simulink model "das_evolution"  (R2026a)
settings: Solver=VariableStepAuto
undefined symbols (not defined in the file): att, B_cell, f_v, g_cir, g_edfa, g_vib, k_lo, k_sig, p_frame, P_laser, Phi0, r, R_pd, Ts_slow, var_phL
settings Model: Creator=aljou  LastModifiedBy=aljou

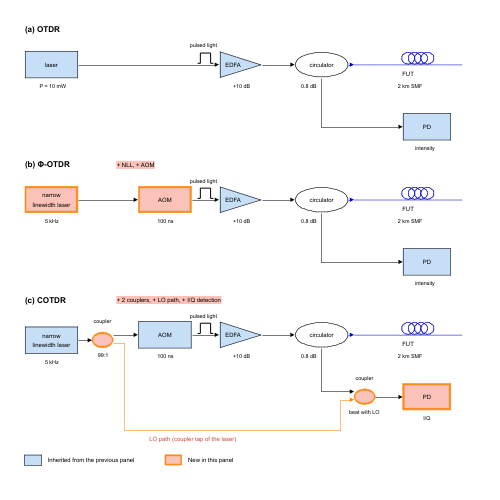
[thumbnail: Simulink's stored preview of the top-level diagram]
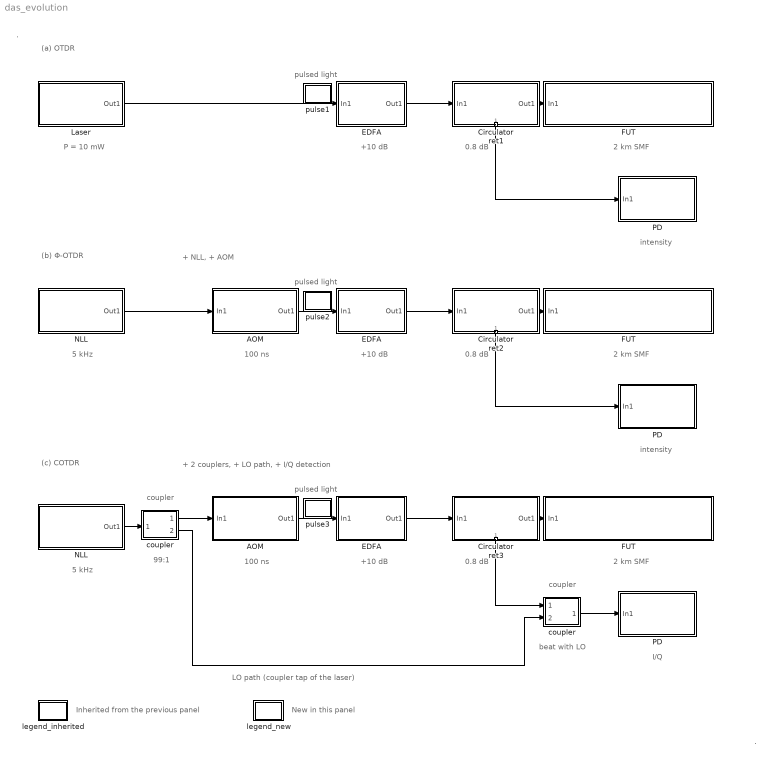
== system das_evolution ==
  note: (a) OTDR
  note: P = 10 mW
  note: +10 dB
  note: 2 km SMF
  note: 0.8 dB
  note: intensity
  note: pulsed light
  note: (b) Φ-OTDR
  note: + NLL, + AOM
  note: 5 kHz
  note: 100 ns
  note: +10 dB
  note: 2 km SMF
  note: 0.8 dB
  note: intensity
  note: pulsed light
  note: (c) COTDR
  note: + 2 couplers, + LO path, + I/Q detection
  note: 99:1
  note: 5 kHz
  note: coupler
  note: 100 ns
  note: +10 dB
  note: 2 km SMF
  note: 0.8 dB
  note: beat with LO
  note: coupler
  note: I/Q
  note: pulsed light
  note: LO path (coupler tap of the laser)
  note: Inherited from the previous panel
  note: New in this panel
  note: .
  note: .
  "AOM        " : Subsystem
      mask Display: patch([0.01 0.99 0.99 0.01],[0.01 0.01 0.99 0.99],[0.98 0.55 0.10]);patch([0.0492 0.9508 0.9508 0.0492],[0.0884 0.0884 0.9116 0.9116],[0.98 0.76 0.72]);color('black');text(0.5,0.5,'AOM','horizontalAlignment','center','verticalAlignment','middle');
  "AOM                 " : Subsystem
      mask Display: patch([0.01 0.99 0.99 0.01],[0.01 0.01 0.99 0.99],[0.78 0.87 0.97]);color('black');plot([0.01 0.99 0.99 0.01 0.01],[0.01 0.01 0.99 0.99 0.01]);color('black');text(0.5,0.5,'AOM','horizontalAlignment','center','verticalAlignment','middle');
  "Circulator  " : Subsystem
      mask Display: patch(0.5+0.49*cos(linspace(0,2*pi,61)),0.5+0.46*sin(linspace(0,2*pi,61)),[1 1 1]);color('black');plot(0.5+0.49*cos(linspace(0,2*pi,61)),0.5+0.46*sin(linspace(0,2*pi,61)));color('black');text(0.5,0.5,'circulator','horizontalAlignment','center','verticalAlignment','middle');
  "Circulator          " : Subsystem
      mask Display: patch(0.5+0.49*cos(linspace(0,2*pi,61)),0.5+0.46*sin(linspace(0,2*pi,61)),[1 1 1]);color('black');plot(0.5+0.49*cos(linspace(0,2*pi,61)),0.5+0.46*sin(linspace(0,2*pi,61)));color('black');text(0.5,0.5,'circulator','horizontalAlignment','center','verticalAlignment','middle');
  "Circulator                   " : Subsystem
      mask Display: patch(0.5+0.49*cos(linspace(0,2*pi,61)),0.5+0.46*sin(linspace(0,2*pi,61)),[1 1 1]);color('black');plot(0.5+0.49*cos(linspace(0,2*pi,61)),0.5+0.46*sin(linspace(0,2*pi,61)));color('black');text(0.5,0.5,'circulator','horizontalAlignment','center','verticalAlignment','middle');
  "EDFA " : Subsystem
      mask Display: patch([0.02 0.02 0.98],[0.02 0.98 0.5],[0.78 0.87 0.97]);color('black');plot([0.02 0.02 0.98 0.02],[0.02 0.98 0.5 0.02]);color('black');text(0.33,0.5,'EDFA','horizontalAlignment','center','verticalAlignment','middle');
  "EDFA         " : Subsystem
      mask Display: patch([0.02 0.02 0.98],[0.02 0.98 0.5],[0.78 0.87 0.97]);color('black');plot([0.02 0.02 0.98 0.02],[0.02 0.98 0.5 0.02]);color('black');text(0.33,0.5,'EDFA','horizontalAlignment','center','verticalAlignment','middle');
  "EDFA                  " : Subsystem
      mask Display: patch([0.02 0.02 0.98],[0.02 0.98 0.5],[0.78 0.87 0.97]);color('black');plot([0.02 0.02 0.98 0.02],[0.02 0.98 0.5 0.02]);color('black');text(0.33,0.5,'EDFA','horizontalAlignment','center','verticalAlignment','middle');
  "FUT   " : Subsystem
      mask Display: color('blue');plot([0 1],[0.5 0.5]);plot(0.5+0.06*cos(linspace(0,2*pi,61)),0.74+0.22*sin(linspace(0,2*pi,61)));plot(0.56+0.06*cos(linspace(0,2*pi,61)),0.74+0.22*sin(linspace(0,2*pi,61)));plot(0.62+0.06*cos(linspace(0,2*pi,61)),0.74+0.22*sin(linspace(0,2*pi,61)));plot(0.68+0.06*cos(linspace(0,2*pi,61)),0.74+0.22*sin(linspace(0,2*pi,61)));color('black');text(0.5,0.16,'FUT','horizontalAlignment','center','verticalAlignment','middle');
  "FUT           " : Subsystem
      mask Display: color('blue');plot([0 1],[0.5 0.5]);plot(0.5+0.06*cos(linspace(0,2*pi,61)),0.74+0.22*sin(linspace(0,2*pi,61)));plot(0.56+0.06*cos(linspace(0,2*pi,61)),0.74+0.22*sin(linspace(0,2*pi,61)));plot(0.62+0.06*cos(linspace(0,2*pi,61)),0.74+0.22*sin(linspace(0,2*pi,61)));plot(0.68+0.06*cos(linspace(0,2*pi,61)),0.74+0.22*sin(linspace(0,2*pi,61)));color('black');text(0.5,0.16,'FUT','horizontalAlignment','center','verticalAlignment','middle');
  "FUT                    " : Subsystem
      mask Display: color('blue');plot([0 1],[0.5 0.5]);plot(0.5+0.06*cos(linspace(0,2*pi,61)),0.74+0.22*sin(linspace(0,2*pi,61)));plot(0.56+0.06*cos(linspace(0,2*pi,61)),0.74+0.22*sin(linspace(0,2*pi,61)));plot(0.62+0.06*cos(linspace(0,2*pi,61)),0.74+0.22*sin(linspace(0,2*pi,61)));plot(0.68+0.06*cos(linspace(0,2*pi,61)),0.74+0.22*sin(linspace(0,2*pi,61)));color('black');text(0.5,0.16,'FUT','horizontalAlignment','center','verticalAlignment','middle');
  Laser : Subsystem
      mask Display: patch([0.01 0.99 0.99 0.01],[0.01 0.01 0.99 0.99],[0.78 0.87 0.97]);color('black');plot([0.01 0.99 0.99 0.01 0.01],[0.01 0.01 0.99 0.99 0.01]);color('black');text(0.5,0.5,'laser','horizontalAlignment','center','verticalAlignment','middle');
  "NLL       " : Subsystem
      mask Display: patch([0.01 0.99 0.99 0.01],[0.01 0.01 0.99 0.99],[0.98 0.55 0.10]);patch([0.0492 0.9508 0.9508 0.0492],[0.0884 0.0884 0.9116 0.9116],[0.98 0.76 0.72]);color('black');text(0.5,0.67,'narrow','horizontalAlignment','center','verticalAlignment','middle');color('black');text(0.5,0.33,'linewidth laser','horizontalAlignment','center','verticalAlignment','middle');
  "NLL                " : Subsystem
      mask Display: patch([0.01 0.99 0.99 0.01],[0.01 0.01 0.99 0.99],[0.78 0.87 0.97]);color('black');plot([0.01 0.99 0.99 0.01 0.01],[0.01 0.01 0.99 0.99 0.01]);color('black');text(0.5,0.67,'narrow','horizontalAlignment','center','verticalAlignment','middle');color('black');text(0.5,0.33,'linewidth laser','horizontalAlignment','center','verticalAlignment','middle');
  "PD    " : Subsystem
      mask Display: patch([0.01 0.99 0.99 0.01],[0.01 0.01 0.99 0.99],[0.78 0.87 0.97]);color('black');plot([0.01 0.99 0.99 0.01 0.01],[0.01 0.01 0.99 0.99 0.01]);color('black');text(0.5,0.5,'PD','horizontalAlignment','center','verticalAlignment','middle');
  "PD            " : Subsystem
      mask Display: patch([0.01 0.99 0.99 0.01],[0.01 0.01 0.99 0.99],[0.78 0.87 0.97]);color('black');plot([0.01 0.99 0.99 0.01 0.01],[0.01 0.01 0.99 0.99 0.01]);color('black');text(0.5,0.5,'PD','horizontalAlignment','center','verticalAlignment','middle');
  "PD                      " : Subsystem
      mask Display: patch([0.01 0.99 0.99 0.01],[0.01 0.01 0.99 0.99],[0.98 0.55 0.10]);patch([0.0492 0.9508 0.9508 0.0492],[0.0884 0.0884 0.9116 0.9116],[0.98 0.76 0.72]);color('black');text(0.5,0.5,'PD','horizontalAlignment','center','verticalAlignment','middle');
  "coupler               " : Subsystem
      mask Display: patch(0.5+0.49*cos(linspace(0,2*pi,61)),0.41935+0.46*sin(linspace(0,2*pi,61)),[0.98 0.55 0.10]);patch(0.5+0.422*cos(linspace(0,2*pi,61)),0.41935+0.34*sin(linspace(0,2*pi,61)),[0.98 0.76 0.72]);
  "coupler                     " : Subsystem
      mask Display: patch(0.5+0.49*cos(linspace(0,2*pi,61)),0.41935+0.46*sin(linspace(0,2*pi,61)),[0.98 0.55 0.10]);patch(0.5+0.422*cos(linspace(0,2*pi,61)),0.41935+0.34*sin(linspace(0,2*pi,61)),[0.98 0.76 0.72]);
  legend_inherited : Subsystem
      mask Display: patch([0.01 0.99 0.99 0.01],[0.01 0.01 0.99 0.99],[0.78 0.87 0.97]);color('black');plot([0.01 0.99 0.99 0.01 0.01],[0.01 0.01 0.99 0.99 0.01]);
  legend_new : Subsystem
      mask Display: patch([0.01 0.99 0.99 0.01],[0.01 0.01 0.99 0.99],[0.98 0.55 0.10]);patch([0.108 0.892 0.892 0.108],[0.1668 0.1668 0.8332 0.8332],[0.98 0.76 0.72]);
  pulse1 : Subsystem
      mask Display: color('black');plot([0.02 0.2 0.2 0.8 0.8 0.98],[0.04 0.04 0.96 0.96 0.04 0.04]);
  pulse2 : Subsystem
      mask Display: color('black');plot([0.02 0.2 0.2 0.8 0.8 0.98],[0.04 0.04 0.96 0.96 0.04 0.04]);
  pulse3 : Subsystem
      mask Display: color('black');plot([0.02 0.2 0.2 0.8 0.8 0.98],[0.04 0.04 0.96 0.96 0.04 0.04]);
  ret1 : Subsystem
  ret2 : Subsystem
  ret3 : Subsystem
  wires:
  Laser/1(Out1) -> "EDFA "/1(In1)
  "EDFA "/1(Out1) -> "Circulator  "/1(In1)
  "Circulator  "/1(Out1) -> "FUT   "/1(In1)
  ret1/1(Out1) -> "PD    "/1(In1)
  "NLL       "/1(Out1) -> "AOM        "/1(In1)
  "AOM        "/1(Out1) -> "EDFA         "/1(In1)
  "EDFA         "/1(Out1) -> "Circulator          "/1(In1)
  "Circulator          "/1(Out1) -> "FUT           "/1(In1)
  ret2/1(Out1) -> "PD            "/1(In1)
  "NLL                "/1(Out1) -> "coupler               "/1(In1)
  "coupler               "/1(Out1) -> "AOM                 "/1(In1)
  "AOM                 "/1(Out1) -> "EDFA                  "/1(In1)
  "EDFA                  "/1(Out1) -> "Circulator                   "/1(In1)
  "Circulator                   "/1(Out1) -> "FUT                    "/1(In1)
  ret3/1(Out1) -> "coupler                     "/1(In1)
  "coupler                     "/1(Out1) -> "PD                      "/1(In1)
  "coupler               "/2(Out2) -> "coupler                     "/2(In2)

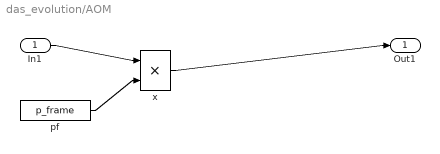
== system das_evolution/AOM         ==
  In1 : Inport
  pf : Constant  Value=p_frame  VectorParams1D=off  SampleTime=Ts_slow
  x : Product  Inputs=**
  Out1 : Outport
  wires:
  In1/1 -> x/1
  pf/1 -> x/2
  x/1 -> Out1/1

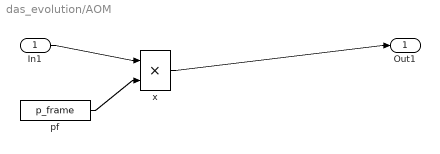
== system das_evolution/AOM                  ==
  In1 : Inport
  pf : Constant  Value=p_frame  VectorParams1D=off  SampleTime=Ts_slow
  x : Product  Inputs=**
  Out1 : Outport
  wires:
  In1/1 -> x/1
  pf/1 -> x/2
  x/1 -> Out1/1

== system das_evolution/Circulator   ==
  In1 : Inport
  g : Gain  Gain=g_cir
  Out1 : Outport
  wires:
  In1/1 -> g/1
  g/1 -> Out1/1

== system das_evolution/Circulator           ==
  In1 : Inport
  g : Gain  Gain=g_cir
  Out1 : Outport
  wires:
  In1/1 -> g/1
  g/1 -> Out1/1

== system das_evolution/Circulator                    ==
  In1 : Inport
  g : Gain  Gain=g_cir
  Out1 : Outport
  wires:
  In1/1 -> g/1
  g/1 -> Out1/1

== system das_evolution/EDFA  ==
  In1 : Inport
  g : Gain  Gain=g_edfa
  Out1 : Outport
  wires:
  In1/1 -> g/1
  g/1 -> Out1/1

== system das_evolution/EDFA          ==
  In1 : Inport
  g : Gain  Gain=g_edfa
  Out1 : Outport
  wires:
  In1/1 -> g/1
  g/1 -> Out1/1

== system das_evolution/EDFA                   ==
  In1 : Inport
  g : Gain  Gain=g_edfa
  Out1 : Outport
  wires:
  In1/1 -> g/1
  g/1 -> Out1/1

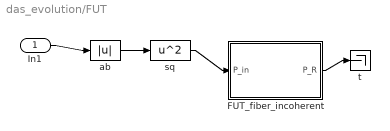
== system das_evolution/FUT    ==
  In1 : Inport
  FUT_fiber_incoherent : MATLAB Function  TreatAsAtomicUnit=on
  ab : Abs  SaturateOnIntegerOverflow=off
  sq : Math  Operator=square
  t : Terminator
  wires:
  In1/1 -> ab/1
  ab/1 -> sq/1
  sq/1 -> FUT_fiber_incoherent/1(P_in)
  FUT_fiber_incoherent/1(P_R) -> t/1

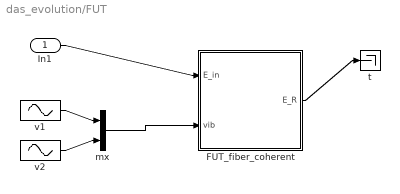
== system das_evolution/FUT            ==
  In1 : Inport
  FUT_fiber_coherent : MATLAB Function  TreatAsAtomicUnit=on
  mx : Mux  Inputs=2
  t : Terminator
  v1 : Sin  Amplitude=Phi0(1)  Frequency=2*pi*f_v(1)  SampleTime=Ts_slow
  v2 : Sin  Amplitude=Phi0(2)  Frequency=2*pi*f_v(2)  SampleTime=Ts_slow
  wires:
  v1/1 -> mx/1
  v2/1 -> mx/2
  In1/1 -> FUT_fiber_coherent/1(E_in)
  mx/1 -> FUT_fiber_coherent/2(vib)
  FUT_fiber_coherent/1(E_R) -> t/1

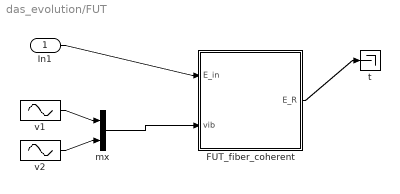
== system das_evolution/FUT                     ==
  In1 : Inport
  FUT_fiber_coherent : MATLAB Function  TreatAsAtomicUnit=on
  mx : Mux  Inputs=2
  t : Terminator
  v1 : Sin  Amplitude=Phi0(1)  Frequency=2*pi*f_v(1)  SampleTime=Ts_slow
  v2 : Sin  Amplitude=Phi0(2)  Frequency=2*pi*f_v(2)  SampleTime=Ts_slow
  wires:
  v1/1 -> mx/1
  v2/1 -> mx/2
  In1/1 -> FUT_fiber_coherent/1(E_in)
  mx/1 -> FUT_fiber_coherent/2(vib)
  FUT_fiber_coherent/1(E_R) -> t/1

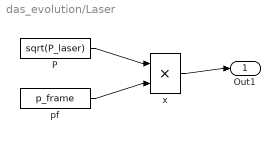
== system das_evolution/Laser ==
  P : Constant  Value=sqrt(P_laser)  SampleTime=Ts_slow
  pf : Constant  Value=p_frame  VectorParams1D=off  SampleTime=Ts_slow
  x : Product  Inputs=**
  Out1 : Outport
  wires:
  P/1 -> x/1
  pf/1 -> x/2
  x/1 -> Out1/1

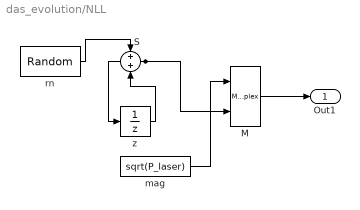
== system das_evolution/NLL        ==
  M : MagnitudeAngleToComplex
  S : Sum
  mag : Constant  Value=sqrt(P_laser)  SampleTime=Ts_slow
  rn : RandomNumber  Variance=var_phL  SampleTime=Ts_slow
  z : UnitDelay  SampleTime=Ts_slow
  Out1 : Outport
  wires:
  rn/1 -> S/1
  S/1 -> z/1, M/2
  z/1 -> S/2
  mag/1 -> M/1
  M/1 -> Out1/1

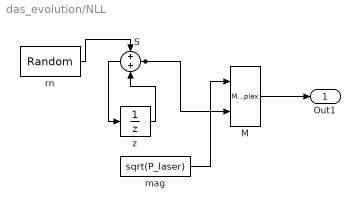
== system das_evolution/NLL                 ==
  M : MagnitudeAngleToComplex
  S : Sum
  mag : Constant  Value=sqrt(P_laser)  SampleTime=Ts_slow
  rn : RandomNumber  Variance=var_phL  SampleTime=Ts_slow
  z : UnitDelay  SampleTime=Ts_slow
  Out1 : Outport
  wires:
  rn/1 -> S/1
  S/1 -> z/1, M/2
  z/1 -> S/2
  mag/1 -> M/1
  M/1 -> Out1/1

== system das_evolution/PD     ==
  In1 : Inport
  g : Gain  Gain=R_pd
  t : Terminator
  wires:
  In1/1 -> g/1
  g/1 -> t/1

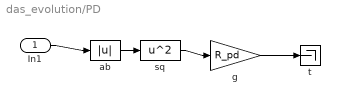
== system das_evolution/PD             ==
  In1 : Inport
  ab : Abs  SaturateOnIntegerOverflow=off
  g : Gain  Gain=R_pd
  sq : Math  Operator=square
  t : Terminator
  wires:
  In1/1 -> ab/1
  ab/1 -> sq/1
  sq/1 -> g/1
  g/1 -> t/1

== system das_evolution/PD                       ==
  In1 : Inport
  g : Gain  Gain=R_pd
  t : Terminator
  wires:
  In1/1 -> g/1
  g/1 -> t/1

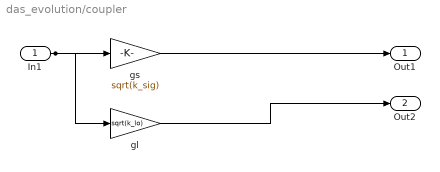
== system das_evolution/coupler                ==
  In1 : Inport
  gl : Gain  Gain=sqrt(k_lo)
  gs : Gain  Gain=sqrt(k_sig)
  Out1 : Outport
  Out2 : Outport  Port=2
  wires:
  In1/1 -> gs/1, gl/1
  gs/1 -> Out1/1
  gl/1 -> Out2/1

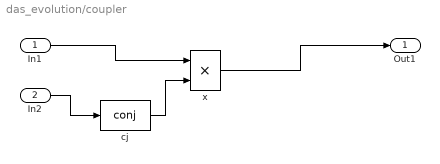
== system das_evolution/coupler                      ==
  In1 : Inport
  In2 : Inport  Port=2
  cj : Math  Operator=conj
  x : Product  Inputs=**
  Out1 : Outport
  wires:
  In1/1 -> x/1
  In2/1 -> cj/1
  cj/1 -> x/2
  x/1 -> Out1/1

== system das_evolution/legend_inherited ==

== system das_evolution/legend_new ==

== system das_evolution/pulse1 ==

== system das_evolution/pulse2 ==

== system das_evolution/pulse3 ==

== system das_evolution/ret1 ==
  c : Constant
  Out1 : Outport
  wires:
  c/1 -> Out1/1

== system das_evolution/ret2 ==
  c : Constant
  Out1 : Outport
  wires:
  c/1 -> Out1/1

== system das_evolution/ret3 ==
  c : Constant
  Out1 : Outport
  wires:
  c/1 -> Out1/1

== matlab function das_evolution/FUT           /FUT_fiber_coherent ==
  data: E_in input; E_R output; vib input; r parameter; att parameter; g_vib parameter
function E_R = fiber_coherent(E_in, vib, r, att, g_vib)
%FIBER_COHERENT  FUT block for Phi-OTDR and COTDR (coherent laser).
%  Paste this into a MATLAB Function block named "FUT (coherent)".
%  Ports and Data Manager settings (set Size explicitly, it avoids dimension errors):
%    E_in  : input,  Size [Ns 1], Complexity complex  (probe frame after EDFA + circulator)
%    vib   : input,  Size [K 1] (or [1 K] from the Mux), real  (vibration phase of each event)
%    r     : PARAMETER (Nz x 1 complex), att : PARAMETER (Nz x 1), g_vib : PARAMETER (Nz x K)
%    E_R   : output, Size [Ns 1], Complexity complex
%
%  Model (Shang 2022, Eq. 4): the received field is the sum of the echoes of
%  all scatterers. Each fibre cell is one scatterer, delayed by its round trip
%  (one sample per cell), so the sum becomes a convolution of the probe with
%  the fibre impulse response h.  A vibration adds a phase to every cell at
%  and beyond the disturbed section.

phi = g_vib * vib(:);                    % Nz x 1 extra phase [rad]  (vib(:) forces a column)
h   = r .* att .* exp(1j*phi);           % fibre impulse response
y   = conv(E_in, h);                     % coherent sum of all echoes
E_R = y(1:numel(E_in));
end

== matlab function das_evolution/FUT   /FUT_fiber_incoherent ==
  data: P_in input; P_R output; B_cell parameter; att parameter
function P_R = fiber_incoherent(P_in, B_cell, att)
%FIBER_INCOHERENT  FUT block for conventional OTDR (low-coherence source).
%  Paste this into a MATLAB Function block named "FUT (incoherent)".
%    P_in   : input,  Size [Ns 1], real   (probe POWER frame = |E|^2)
%    B_cell : PARAMETER (scalar)          (backscattered power fraction per cell)
%    att    : PARAMETER (Nz x 1)          (same as the coherent block)
%    P_R    : output, Size [Ns 1], real   (backscattered POWER)
%
%  With a low-coherence source the echoes do not interfere: powers add, not
%  fields. The vibration phase therefore has no effect on the trace — this is
%  exactly why conventional OTDR cannot sense vibration (Shang 2022, Sec. 2.2).
%
%  Change vs the original: the power response uses the AVERAGE scattering power
%  B_cell instead of the random |r|^2. A low-coherence source averages the
%  speckle away, so the trace is a smooth line (slope = 2*alpha).

h   = B_cell .* att.^2;                  % power impulse response (round trip)
y   = conv(P_in, h);
P_R = y(1:numel(P_in));
end

== matlab function das_evolution/FUT                    /FUT_fiber_coherent ==
  data: E_in input; E_R output; vib input; r parameter; att parameter; g_vib parameter
function E_R = fiber_coherent(E_in, vib, r, att, g_vib)
%FIBER_COHERENT  FUT block for Phi-OTDR and COTDR (coherent laser).
%  Paste this into a MATLAB Function block named "FUT (coherent)".
%  Ports and Data Manager settings (set Size explicitly, it avoids dimension errors):
%    E_in  : input,  Size [Ns 1], Complexity complex  (probe frame after EDFA + circulator)
%    vib   : input,  Size [K 1] (or [1 K] from the Mux), real  (vibration phase of each event)
%    r     : PARAMETER (Nz x 1 complex), att : PARAMETER (Nz x 1), g_vib : PARAMETER (Nz x K)
%    E_R   : output, Size [Ns 1], Complexity complex
%
%  Model (Shang 2022, Eq. 4): the received field is the sum of the echoes of
%  all scatterers. Each fibre cell is one scatterer, delayed by its round trip
%  (one sample per cell), so the sum becomes a convolution of the probe with
%  the fibre impulse response h.  A vibration adds a phase to every cell at
%  and beyond the disturbed section.

phi = g_vib * vib(:);                    % Nz x 1 extra phase [rad]  (vib(:) forces a column)
h   = r .* att .* exp(1j*phi);           % fibre impulse response
y   = conv(E_in, h);                     % coherent sum of all echoes
E_R = y(1:numel(E_in));
end
